simulink model "afe"  (R2026a)
settings: Solver=ode23tb  StopTime=simlength  FixedStep=tc  MaxStep=glb_time.tc
values from neighbouring files (symbols this model uses):
  afe_ctrl = ctrl_afe_setup(glb_time.ts_afe, grid_emu.omega_grid_nom)    [init_model.m]
  afe_pwm_phase_shift_mod1 = 0    [init_model.m]
  CTRPIFF_CLIP_RELEASE = 0.001    [init_model.m]
  glb_time = timing_setup(fpwm_afe, trgo_afe, fpwm_inv, trgo_inv, fpwm_single_phase_inv, trgo_single_phase_inv, fpwm_dab, trgo_dab,      fpwm_psfbc, trgo_psfbc, fpwm_isop_rail, trgo_isop_rail, fpwm_cllc, trgo_cllc, t_measure, tc_factor, tc_decimation, delay_pwm, dead_time_afe,      dead_time_inv, dead_time_single_phase_inv, dead_time_dab, dead_time_psfbc, dead_time_isop_rail, dead_time_cllc)    [init_model.m]
  grid_emu = grid_three_phase_emulator('Dyn11', delta_star, grid_nominal_power, application_voltage, us1, us2, fgrid,                  eq_grid_inductance, eq_grid_resistance, eta, ucc, i1m, p_iron, n1, n2, core_area, core_length, mur,                  up_xi_pu_ref, up_eta_pu_ref, un_xi_pu_ref, un_eta_pu_ref)    [init_model.m]
  heatsink = liquid_cooled_plate_2kw_setup(weight, no_weight, cp_al, heat_capacity_hs, thermal_conductivity_al,      Rth_switch_HA, Rth_mosfet_HA, Rth_diode_HA, Tambient, DThs_init)    [init_model.m]
  ki_align = 18    [init_model.m]
  kp_align = 0.25    [init_model.m]
  lim_down_align = -0.05    [init_model.m]
  lim_up_align = 0.05    [init_model.m]
  psm_ctrl = ctrl_pmsm_setup(glb_time.ts_inv, psm.omega_bez, u_psm_scale, psm.Jm_norm)    [init_model.m]
  Tambient = 40    [init_model.m]
  time_gain_afe_module_1 = 1.0002    [init_model.m]
  time_gain_inv_module_2 = 1.001    [init_model.m]
  u_cm_comp_mod1 = 0    [init_model.m]
undefined symbols (not defined in the file or in its folder): hwdata, igbt, magnitude
libraries: fl_lib x166, nesl_utility x91, igbt_simple_2th_lib x4, single_phase_transformer_lib x3, mos_simple_2th_lib x2, discrete_time_low_pass_filter x1, threephase_inductor_lib x1, dclink_for_two_levels x1, three_phase_pwm_modulator x1, three_phase_voltage_with_frt_emulator x1
(part 5 of 7)

== system afe/afe/afe_dq_mod1/AFE_control/afe_control/grid_voltage_phase_lock_loops/dq_pll_ccaller/first_harmonic_tracker_phase_w ==
  u : Inport
  Bus Selector : BusSelector  OutputSignals=output_pu_hat
  C Caller : CCaller  FunctionName=first_harmonic_tracker_process_simulink  PortSpecificationStruct="%)30     .    B \\   8    (     @         %    \"     D    !     0         %  0 \"0    $    _    07)G3F%M90  4&]R=$YA;64 4V-O<&4     26YD97@     5'EP90      4VEZ90      27-';&]B86P   X    P    !@    @    $          4    (     0    ,    !         !   P!O=70 #@   #     &    \"     0         !0    @    !     P    $         $  # &]U=  .    .     8    (    !          %    \"     $    &     0         0  ...(+4988 chars)"
  Constant : Constant  Value=glb_time.ts_afe
  Constant1 : Constant  Value=4
  Constant4 : Constant  Value=afe_ctrl.fht_grid.omega_fht
  Constant5 : Constant  Value=afe_ctrl.fht_grid.delta_fht
  Constant6 : Constant  Value=afe_ctrl.fht_grid.Ld_fht(1)
  Constant7 : Constant  Value=afe_ctrl.fht_grid.Ld_fht(2)
  Data Type Conversion{1..2,6..9} (6 alike) : DataTypeConversion  OutDataTypeStr=single  SaturateOnIntegerOverflow=off  RndMeth=Floor
  Data Type Conversion3 : DataTypeConversion  OutDataTypeStr=uint8  SaturateOnIntegerOverflow=off  RndMeth=Floor
  Data Type Conversion4 : DataTypeConversion  OutDataTypeStr=double  SaturateOnIntegerOverflow=off  RndMeth=Floor
  Data Type Conversion5 : DataTypeConversion  OutDataTypeStr=uint8  SaturateOnIntegerOverflow=off  RndMeth=Floor
  Step : Step  Time=0.0125  InitialValue=1  FinalValue=0
  u_hat : Outport
  wires:
  Data Type Conversion4/1 -> u_hat/1
  Data Type Conversion3/1 -> C Caller/1
  Data Type Conversion1/1 -> C Caller/3
  Data Type Conversion2/1 -> C Caller/2
  C Caller/1 -> Bus Selector/1
  Bus Selector/1 -> Data Type Conversion4/1  "<output_pu_hat>"
  Step/1 -> Data Type Conversion3/1
  u/1 -> Data Type Conversion2/1
  Constant/1 -> Data Type Conversion1/1
  Constant1/1 -> Data Type Conversion5/1
  Constant4/1 -> Data Type Conversion6/1
  Constant6/1 -> Data Type Conversion8/1
  Constant7/1 -> Data Type Conversion9/1
  Constant5/1 -> Data Type Conversion7/1
  Data Type Conversion5/1 -> C Caller/8
  Data Type Conversion6/1 -> C Caller/4
  Data Type Conversion7/1 -> C Caller/5
  Data Type Conversion8/1 -> C Caller/6
  Data Type Conversion9/1 -> C Caller/7

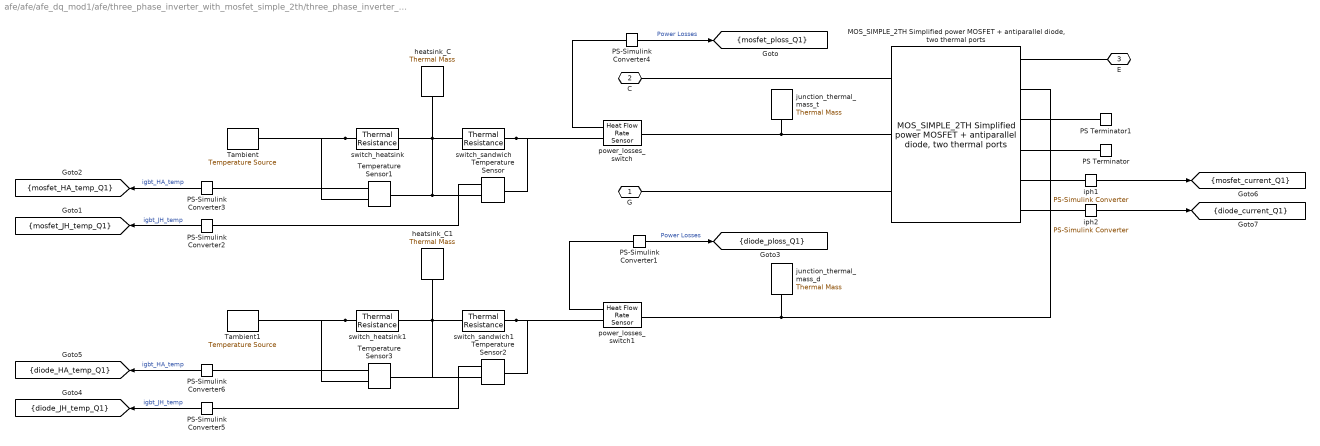
== system afe/afe/afe_dq_mod1/afe/three_phase_inverter_with_mosfet_simple_2th/three_phase_inverter_with_mosfet_simple_2th/mosfet_simple_1/MOSFET_simple ==
  "MOS_SIMPLE_2TH Simplified power MOSFET + antiparallel diode, two thermal ports" : mos_simple_2th_lib/MOS_SIMPLE_2TH Simplified power MOSFET + antiparallel diode, two thermal ports  Rds_on=rds_on_m Ohm  alpha_R=0 1/K  Tj_ref=398.15 K  Roff=1e7 Ohm  Vf=1.0 V  Rd=2.5e-3 Ohm  two_die=1  Eon_ref=Eon_m J  Eoff_ref=Eoff_m J  Err_ref=Err_m J  Iref=Ic_ref_m A  Vref=Vdc_ref_m V  ki=1  kv=1  Vth_off=50 V  Vth_on=25 V  V_sm=10 V  tau_s=100e-9 s  tau_v=10e-6 s  tau_p=50e-6 s  i_eps=1e-3 A  v_eps=1e-3 V  v_specify=off  v_priority=None  v=0 V  v_nominal_specify=off  v_nominal_value=1  v_nominal_unit=V  i_specify=off  i_priority=None  i=0 A  i_nominal_specify=off  i_nominal_value=1  i_nominal_unit=A  ich_specify=off  ich_priority=None  ich=0 A  ich_nominal_specify=off  ich_nominal_value=1  ich_nominal_unit=A  ichp_specify=off  ichp_priority=None  ichp=0 A  ichp_nominal_specify=off  ichp_nominal_value=1  ichp_nominal_unit=A  idio_specify=off  idio_priority=None  idio=0 A  idio_nominal_specify=off  idio_nominal_value=1  idio_nominal_unit=A  vfd_specify=off  vfd_priority=None  vfd=0 V  vfd_nominal_specify=off  vfd_nominal_value=1  vfd_nominal_unit=V  ith_specify=off  ith_priority=None  ith=0 A  ith_nominal_specify=off  ith_nominal_value=1  ith_nominal_unit=A  idh_specify=off  idh_priority=None  idh=0 A  idh_nominal_specify=off  idh_nominal_value=1  idh_nominal_unit=A  vbl_specify=off  vbl_priority=None  vbl=600 V  vbl_nominal_specify=off  vbl_nominal_value=1  vbl_nominal_unit=V  hb_specify=off  hb_priority=None  hb=0  hb_nominal_specify=off  hb_nominal_value=1  hb_nominal_unit=1  Gch_specify=off  Gch_priority=None  Gch=0 S  Gch_nominal_specify=off  Gch_nominal_value=1  Gch_nominal_unit=S  Rds_specify=off  Rds_priority=None  Rds=1e-3 Ohm  Rds_nominal_specify=off  Rds_nominal_value=1  Rds_nominal_unit=Ohm  xr_specify=off  xr_priority=None  xr=1  xr_nominal_specify=off  xr_nominal_value=1  xr_nominal_unit=1  Eot_specify=off  Eot_priority=None  Eot=0 J  Eot_nominal_specify=off  Eot_nominal_value=1  Eot_nominal_unit=J  Eod_specify=off  Eod_priority=None  Eod=0 J  Eod_nominal_specify=off  Eod_nominal_value=1  Eod_nominal_unit=J  Pswt_specify=off  Pswt_priority=None  Pswt=0 W  Pswt_nominal_specify=off  Pswt_nominal_value=1  Pswt_nominal_unit=W  Pswd_specify=off  Pswd_priority=None  Pswd=0 W  Pswd_nominal_specify=off  Pswd_nominal_value=1  Pswd_nominal_unit=W  Pct_specify=off  Pct_priority=None  Pct=0 W  Pct_nominal_specify=off  Pct_nominal_value=1  Pct_nominal_unit=W  Pcd_specify=off  Pcd_priority=None  Pcd=0 W  Pcd_nominal_specify=off  Pcd_nominal_value=1  Pcd_nominal_unit=W  Qt_specify=off  Qt_priority=None  Qt=0 W  Qt_nominal_specify=off  Qt_nominal_value=1  Qt_nominal_unit=W  Qd_specify=off  Qd_priority=None  Qd=0 W  Qd_nominal_specify=off  Qd_nominal_value=1  Qd_nominal_unit=W  Eqt_specify=off  Eqt_priority=None  Eqt=0 J  Eqd_specify=off  Eqd_priority=None  Eqd=0 J
  PS Terminator : fl_lib/Physical Signals/Sinks/PS Terminator
  PS Terminator1 : fl_lib/Physical Signals/Sinks/PS Terminator
  PS-Simulink Converter1 : nesl_utility/PS-Simulink Converter  PhysicalDomain=network_engine_domain  SubClassName=ps_output  LeftPortType=input  RightPortType=output  PseudoPeriodic=off  Frequencies=[]  VectorFormat=1-D array  Unit=J/s  AffineConversion=off
  PS-Simulink Converter{2..3,5..6} (4 alike) : nesl_utility/PS-Simulink Converter  PhysicalDomain=network_engine_domain  SubClassName=ps_output  LeftPortType=input  RightPortType=output  PseudoPeriodic=off  Frequencies=[]  VectorFormat=1-D array  Unit=degC  AffineConversion=off
  PS-Simulink Converter4 : nesl_utility/PS-Simulink Converter  PhysicalDomain=network_engine_domain  SubClassName=ps_output  LeftPortType=input  RightPortType=output  PseudoPeriodic=off  Frequencies=[]  VectorFormat=1-D array  Unit=J/s  AffineConversion=off
  Tambient : fl_lib/Thermal/Thermal Sources/Temperature Source  temperature=Tambient_m degC
  Tambient1 : fl_lib/Thermal/Thermal Sources/Temperature Source  temperature=Tambient_m degC
  Temperature Sensor{,1..3} (4 alike) : fl_lib/Thermal/Thermal Sensors/Temperature Sensor  temperature_measure=foundation.enum.MeasurementReference.difference
  heatsink_C : fl_lib/Thermal/Thermal Elements/Thermal Mass  mass_type=foundation.enum.constant_variable.constant  mass=mass_heatsink_m kg  sp_heat=specific_heat_m J/(K*kg)  mass_min=1e-6 kg  num_ports=foundation.enum.numPorts2.one  m_specify=off  m_priority=High  m=1 kg  m_nominal_specify=off  m_nominal_value=1  m_nominal_unit=kg  T_specify=on  T_priority=High  T=Tambient_m degC  T_nominal_specify=off  T_nominal_value=1  T_nominal_unit=K  Q_specify=off  Q_priority=High  Q=0 W  Q_nominal_specify=off  Q_nominal_value=1  Q_nominal_unit=W
  heatsink_C1 : fl_lib/Thermal/Thermal Elements/Thermal Mass  mass_type=foundation.enum.constant_variable.constant  mass=mass_heatsink_m kg  sp_heat=specific_heat_m J/(K*kg)  mass_min=1e-6 kg  num_ports=foundation.enum.numPorts2.one  m_specify=off  m_priority=High  m=1 kg  m_nominal_specify=off  m_nominal_value=1  m_nominal_unit=kg  T_specify=on  T_priority=High  T=Tambient_m degC  T_nominal_specify=off  T_nominal_value=1  T_nominal_unit=K  Q_specify=off  Q_priority=High  Q=0 W  Q_nominal_specify=off  Q_nominal_value=1  Q_nominal_unit=W
  iph1 : nesl_utility/PS-Simulink Converter  PhysicalDomain=network_engine_domain  SubClassName=ps_output  LeftPortType=input  RightPortType=output  PseudoPeriodic=off  Frequencies=[]  VectorFormat=1-D array  Unit=A  AffineConversion=off
  iph2 : nesl_utility/PS-Simulink Converter  PhysicalDomain=network_engine_domain  SubClassName=ps_output  LeftPortType=input  RightPortType=output  PseudoPeriodic=off  Frequencies=[]  VectorFormat=1-D array  Unit=A  AffineConversion=off
  junction_thermal_mass_d : fl_lib/Thermal/Thermal Elements/Thermal Mass  mass_type=foundation.enum.constant_variable.constant  mass=JunctionTermalMass_m/specific_heat_m kg  sp_heat=specific_heat_m J/(K*kg)  mass_min=1e-6 kg  num_ports=foundation.enum.numPorts2.one  m_specify=off  m_priority=High  m=1 kg  m_nominal_specify=off  m_nominal_value=1  m_nominal_unit=kg  T_specify=on  T_priority=High  T=Tambient_m degC  T_nominal_specify=off  T_nominal_value=1  T_nominal_unit=K  Q_specify=off  Q_priority=High  Q=0 W  Q_nominal_specify=off  Q_nominal_value=1  Q_nominal_unit=W
  junction_thermal_mass_t : fl_lib/Thermal/Thermal Elements/Thermal Mass  mass_type=foundation.enum.constant_variable.constant  mass=JunctionTermalMass_m/specific_heat_m kg  sp_heat=specific_heat_m J/(K*kg)  mass_min=1e-6 kg  num_ports=foundation.enum.numPorts2.one  m_specify=off  m_priority=High  m=1 kg  m_nominal_specify=off  m_nominal_value=1  m_nominal_unit=kg  T_specify=on  T_priority=High  T=Tambient_m degC  T_nominal_specify=off  T_nominal_value=1  T_nominal_unit=K  Q_specify=off  Q_priority=High  Q=0 W  Q_nominal_specify=off  Q_nominal_value=1  Q_nominal_unit=W
  power_losses_switch : fl_lib/Thermal/Thermal Sensors/Heat Flow Rate Sensor
  power_losses_switch1 : fl_lib/Thermal/Thermal Sensors/Heat Flow Rate Sensor
  switch_heatsink : fl_lib/Thermal/Thermal Elements/Thermal Resistance  resistance=rth_switch_HA_m K/W  T_specify=off  T_priority=High  T=0 deltadegC  T_nominal_specify=off  T_nominal_value=1  T_nominal_unit=K  Q_specify=off  Q_priority=None  Q=0 W  Q_nominal_specify=off  Q_nominal_value=1  Q_nominal_unit=W
  switch_heatsink1 : fl_lib/Thermal/Thermal Elements/Thermal Resistance  resistance=rth_diode_HA_m K/W  T_specify=off  T_priority=High  T=0 deltadegC  T_nominal_specify=off  T_nominal_value=1  T_nominal_unit=K  Q_specify=off  Q_priority=None  Q=0 W  Q_nominal_specify=off  Q_nominal_value=1  Q_nominal_unit=W
  switch_sandwich : fl_lib/Thermal/Thermal Elements/Thermal Resistance  resistance=rth_switch_JH_m K/W  T_specify=off  T_priority=High  T=0 degC  T_nominal_specify=off  T_nominal_value=1  T_nominal_unit=K  Q_specify=off  Q_priority=None  Q=0 W  Q_nominal_specify=off  Q_nominal_value=1  Q_nominal_unit=W
  switch_sandwich1 : fl_lib/Thermal/Thermal Elements/Thermal Resistance  resistance=rth_diode_JH_m K/W  T_specify=off  T_priority=High  T=0 degC  T_nominal_specify=off  T_nominal_value=1  T_nominal_unit=K  Q_specify=off  Q_priority=None  Q=0 W  Q_nominal_specify=off  Q_nominal_value=1  Q_nominal_unit=W
  G : PMIOPort  Side=Left
  C : PMIOPort  Port=2  Side=Left
  E : PMIOPort  Port=3  Side=Right
  tag scope: diode_HA_temp_Q1=scoped, diode_JH_temp_Q1=scoped, diode_current_Q1=scoped, diode_ploss_Q1=scoped, mosfet_HA_temp_Q1=scoped, mosfet_JH_temp_Q1=scoped, mosfet_current_Q1=scoped, mosfet_ploss_Q1=scoped
  wires:
  PS-Simulink Converter3/1 -> [mosfet_HA_temp_Q1]  "igbt_HA_temp"
  PS-Simulink Converter4/1 -> [mosfet_ploss_Q1]  "Power Losses"
  PS-Simulink Converter2/1 -> [mosfet_JH_temp_Q1]  "igbt_JH_temp"
  PS-Simulink Converter1/1 -> [diode_ploss_Q1]  "Power Losses"
  PS-Simulink Converter5/1 -> [diode_JH_temp_Q1]  "igbt_JH_temp"
  PS-Simulink Converter6/1 -> [diode_HA_temp_Q1]  "igbt_HA_temp"
  iph1/1 -> [mosfet_current_Q1]
  iph2/1 -> [diode_current_Q1]
  connections:
  Temperature Sensor/RConn2 -- PS-Simulink Converter2/LConn1
  junction_thermal_mass_t/LConn1 -- "MOS_SIMPLE_2TH Simplified power MOSFET + antiparallel diode, two thermal ports"/LConn2 -- power_losses_switch/LConn1
  Temperature Sensor1/RConn2 -- PS-Simulink Converter3/LConn1
  Temperature Sensor1/LConn1 -- Temperature Sensor/RConn1 -- switch_heatsink/LConn1 -- heatsink_C/LConn1 -- switch_sandwich/RConn1
  switch_heatsink/RConn1 -- Tambient/LConn1 -- Temperature Sensor1/RConn1
  switch_sandwich/LConn1 -- power_losses_switch/RConn2 -- Temperature Sensor/LConn1
  "MOS_SIMPLE_2TH Simplified power MOSFET + antiparallel diode, two thermal ports"/RConn1 -- E/RConn1
  "MOS_SIMPLE_2TH Simplified power MOSFET + antiparallel diode, two thermal ports"/LConn1 -- C/RConn1
  "MOS_SIMPLE_2TH Simplified power MOSFET + antiparallel diode, two thermal ports"/LConn3 -- G/RConn1
  switch_heatsink1/LConn1 -- switch_sandwich1/RConn1 -- heatsink_C1/LConn1 -- Temperature Sensor2/RConn1 -- Temperature Sensor3/LConn1
  switch_heatsink1/RConn1 -- Temperature Sensor3/RConn1 -- Tambient1/LConn1
  switch_sandwich1/LConn1 -- Temperature Sensor2/LConn1 -- power_losses_switch1/RConn2
  Temperature Sensor3/RConn2 -- PS-Simulink Converter6/LConn1
  Temperature Sensor2/RConn2 -- PS-Simulink Converter5/LConn1
  power_losses_switch1/LConn1 -- "MOS_SIMPLE_2TH Simplified power MOSFET + antiparallel diode, two thermal ports"/RConn2 -- junction_thermal_mass_d/LConn1
  "MOS_SIMPLE_2TH Simplified power MOSFET + antiparallel diode, two thermal ports"/RConn5 -- iph1/LConn1
  "MOS_SIMPLE_2TH Simplified power MOSFET + antiparallel diode, two thermal ports"/RConn6 -- iph2/LConn1
  "MOS_SIMPLE_2TH Simplified power MOSFET + antiparallel diode, two thermal ports"/RConn3 -- PS Terminator1/LConn1
  "MOS_SIMPLE_2TH Simplified power MOSFET + antiparallel diode, two thermal ports"/RConn4 -- PS Terminator/LConn1
  PS-Simulink Converter4/LConn1 -- power_losses_switch/RConn1
  PS-Simulink Converter1/LConn1 -- power_losses_switch1/RConn1

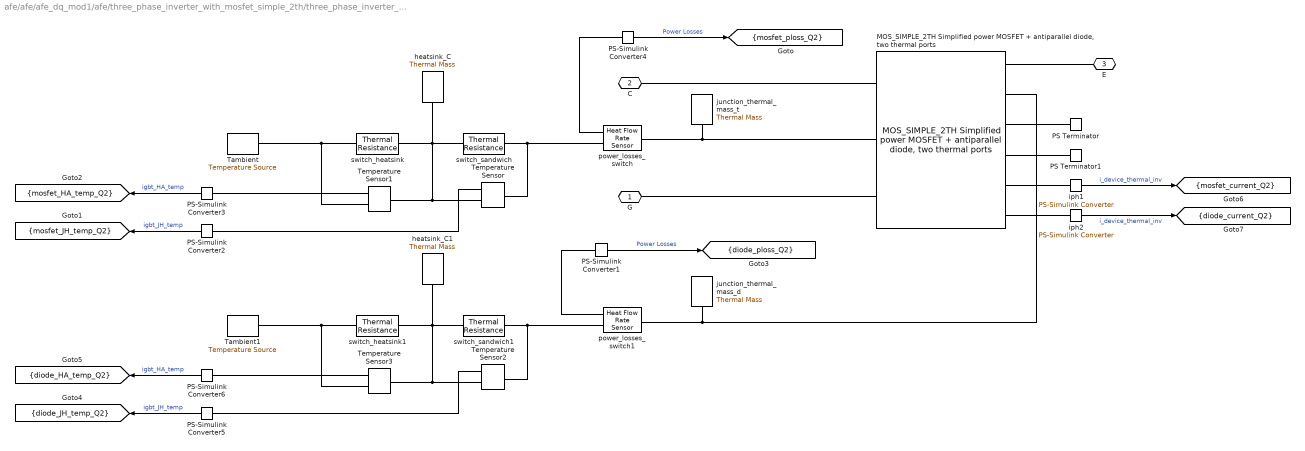
== system afe/afe/afe_dq_mod1/afe/three_phase_inverter_with_mosfet_simple_2th/three_phase_inverter_with_mosfet_simple_2th/mosfet_simple_2/MOSFET_simple ==
  "MOS_SIMPLE_2TH Simplified power MOSFET + antiparallel diode, two thermal ports" : mos_simple_2th_lib/MOS_SIMPLE_2TH Simplified power MOSFET + antiparallel diode, two thermal ports  Rds_on=rds_on_m Ohm  alpha_R=0 1/K  Tj_ref=398.15 K  Roff=1e7 Ohm  Vf=1.0 V  Rd=2.5e-3 Ohm  two_die=1  Eon_ref=Eon_m J  Eoff_ref=Eoff_m J  Err_ref=Err_m J  Iref=Ic_ref_m A  Vref=Vdc_ref_m V  ki=1  kv=1  Vth_off=50 V  Vth_on=25 V  V_sm=10 V  tau_s=100e-9 s  tau_v=10e-6 s  tau_p=50e-6 s  i_eps=1e-3 A  v_eps=1e-3 V  v_specify=off  v_priority=None  v=0 V  v_nominal_specify=off  v_nominal_value=1  v_nominal_unit=V  i_specify=off  i_priority=None  i=0 A  i_nominal_specify=off  i_nominal_value=1  i_nominal_unit=A  ich_specify=off  ich_priority=None  ich=0 A  ich_nominal_specify=off  ich_nominal_value=1  ich_nominal_unit=A  ichp_specify=off  ichp_priority=None  ichp=0 A  ichp_nominal_specify=off  ichp_nominal_value=1  ichp_nominal_unit=A  idio_specify=off  idio_priority=None  idio=0 A  idio_nominal_specify=off  idio_nominal_value=1  idio_nominal_unit=A  vfd_specify=off  vfd_priority=None  vfd=0 V  vfd_nominal_specify=off  vfd_nominal_value=1  vfd_nominal_unit=V  ith_specify=off  ith_priority=None  ith=0 A  ith_nominal_specify=off  ith_nominal_value=1  ith_nominal_unit=A  idh_specify=off  idh_priority=None  idh=0 A  idh_nominal_specify=off  idh_nominal_value=1  idh_nominal_unit=A  vbl_specify=off  vbl_priority=None  vbl=600 V  vbl_nominal_specify=off  vbl_nominal_value=1  vbl_nominal_unit=V  hb_specify=off  hb_priority=None  hb=0  hb_nominal_specify=off  hb_nominal_value=1  hb_nominal_unit=1  Gch_specify=off  Gch_priority=None  Gch=0 S  Gch_nominal_specify=off  Gch_nominal_value=1  Gch_nominal_unit=S  Rds_specify=off  Rds_priority=None  Rds=1e-3 Ohm  Rds_nominal_specify=off  Rds_nominal_value=1  Rds_nominal_unit=Ohm  xr_specify=off  xr_priority=None  xr=1  xr_nominal_specify=off  xr_nominal_value=1  xr_nominal_unit=1  Eot_specify=off  Eot_priority=None  Eot=0 J  Eot_nominal_specify=off  Eot_nominal_value=1  Eot_nominal_unit=J  Eod_specify=off  Eod_priority=None  Eod=0 J  Eod_nominal_specify=off  Eod_nominal_value=1  Eod_nominal_unit=J  Pswt_specify=off  Pswt_priority=None  Pswt=0 W  Pswt_nominal_specify=off  Pswt_nominal_value=1  Pswt_nominal_unit=W  Pswd_specify=off  Pswd_priority=None  Pswd=0 W  Pswd_nominal_specify=off  Pswd_nominal_value=1  Pswd_nominal_unit=W  Pct_specify=off  Pct_priority=None  Pct=0 W  Pct_nominal_specify=off  Pct_nominal_value=1  Pct_nominal_unit=W  Pcd_specify=off  Pcd_priority=None  Pcd=0 W  Pcd_nominal_specify=off  Pcd_nominal_value=1  Pcd_nominal_unit=W  Qt_specify=off  Qt_priority=None  Qt=0 W  Qt_nominal_specify=off  Qt_nominal_value=1  Qt_nominal_unit=W  Qd_specify=off  Qd_priority=None  Qd=0 W  Qd_nominal_specify=off  Qd_nominal_value=1  Qd_nominal_unit=W  Eqt_specify=off  Eqt_priority=None  Eqt=0 J  Eqd_specify=off  Eqd_priority=None  Eqd=0 J
  PS Terminator : fl_lib/Physical Signals/Sinks/PS Terminator
  PS Terminator1 : fl_lib/Physical Signals/Sinks/PS Terminator
  PS-Simulink Converter1 : nesl_utility/PS-Simulink Converter  PhysicalDomain=network_engine_domain  SubClassName=ps_output  LeftPortType=input  RightPortType=output  PseudoPeriodic=off  Frequencies=[]  VectorFormat=1-D array  Unit=J/s  AffineConversion=off
  PS-Simulink Converter{2..3,5..6} (4 alike) : nesl_utility/PS-Simulink Converter  PhysicalDomain=network_engine_domain  SubClassName=ps_output  LeftPortType=input  RightPortType=output  PseudoPeriodic=off  Frequencies=[]  VectorFormat=1-D array  Unit=degC  AffineConversion=off
  PS-Simulink Converter4 : nesl_utility/PS-Simulink Converter  PhysicalDomain=network_engine_domain  SubClassName=ps_output  LeftPortType=input  RightPortType=output  PseudoPeriodic=off  Frequencies=[]  VectorFormat=1-D array  Unit=J/s  AffineConversion=off
  Tambient : fl_lib/Thermal/Thermal Sources/Temperature Source  temperature=Tambient_m degC
  Tambient1 : fl_lib/Thermal/Thermal Sources/Temperature Source  temperature=Tambient_m degC
  Temperature Sensor{,1..3} (4 alike) : fl_lib/Thermal/Thermal Sensors/Temperature Sensor  temperature_measure=foundation.enum.MeasurementReference.difference
  heatsink_C : fl_lib/Thermal/Thermal Elements/Thermal Mass  mass_type=foundation.enum.constant_variable.constant  mass=mass_heatsink_m kg  sp_heat=specific_heat_m J/(K*kg)  mass_min=1e-6 kg  num_ports=foundation.enum.numPorts2.one  m_specify=off  m_priority=High  m=1 kg  m_nominal_specify=off  m_nominal_value=1  m_nominal_unit=kg  T_specify=on  T_priority=High  T=Tambient_m degC  T_nominal_specify=off  T_nominal_value=1  T_nominal_unit=K  Q_specify=off  Q_priority=High  Q=0 W  Q_nominal_specify=off  Q_nominal_value=1  Q_nominal_unit=W
  heatsink_C1 : fl_lib/Thermal/Thermal Elements/Thermal Mass  mass_type=foundation.enum.constant_variable.constant  mass=mass_heatsink_m kg  sp_heat=specific_heat_m J/(K*kg)  mass_min=1e-6 kg  num_ports=foundation.enum.numPorts2.one  m_specify=off  m_priority=High  m=1 kg  m_nominal_specify=off  m_nominal_value=1  m_nominal_unit=kg  T_specify=on  T_priority=High  T=Tambient_m degC  T_nominal_specify=off  T_nominal_value=1  T_nominal_unit=K  Q_specify=off  Q_priority=High  Q=0 W  Q_nominal_specify=off  Q_nominal_value=1  Q_nominal_unit=W
  iph1 : nesl_utility/PS-Simulink Converter  PhysicalDomain=network_engine_domain  SubClassName=ps_output  LeftPortType=input  RightPortType=output  PseudoPeriodic=off  Frequencies=[]  VectorFormat=1-D array  Unit=A  AffineConversion=off
  iph2 : nesl_utility/PS-Simulink Converter  PhysicalDomain=network_engine_domain  SubClassName=ps_output  LeftPortType=input  RightPortType=output  PseudoPeriodic=off  Frequencies=[]  VectorFormat=1-D array  Unit=A  AffineConversion=off
  junction_thermal_mass_d : fl_lib/Thermal/Thermal Elements/Thermal Mass  mass_type=foundation.enum.constant_variable.constant  mass=JunctionTermalMass_m/specific_heat_m kg  sp_heat=specific_heat_m J/(K*kg)  mass_min=1e-6 kg  num_ports=foundation.enum.numPorts2.one  m_specify=off  m_priority=High  m=1 kg  m_nominal_specify=off  m_nominal_value=1  m_nominal_unit=kg  T_specify=on  T_priority=High  T=Tambient_m degC  T_nominal_specify=off  T_nominal_value=1  T_nominal_unit=K  Q_specify=off  Q_priority=High  Q=0 W  Q_nominal_specify=off  Q_nominal_value=1  Q_nominal_unit=W
  junction_thermal_mass_t : fl_lib/Thermal/Thermal Elements/Thermal Mass  mass_type=foundation.enum.constant_variable.constant  mass=JunctionTermalMass_m/specific_heat_m kg  sp_heat=specific_heat_m J/(K*kg)  mass_min=1e-6 kg  num_ports=foundation.enum.numPorts2.one  m_specify=off  m_priority=High  m=1 kg  m_nominal_specify=off  m_nominal_value=1  m_nominal_unit=kg  T_specify=on  T_priority=High  T=Tambient_m degC  T_nominal_specify=off  T_nominal_value=1  T_nominal_unit=K  Q_specify=off  Q_priority=High  Q=0 W  Q_nominal_specify=off  Q_nominal_value=1  Q_nominal_unit=W
  power_losses_switch : fl_lib/Thermal/Thermal Sensors/Heat Flow Rate Sensor
  power_losses_switch1 : fl_lib/Thermal/Thermal Sensors/Heat Flow Rate Sensor
  switch_heatsink : fl_lib/Thermal/Thermal Elements/Thermal Resistance  resistance=rth_switch_HA_m K/W  T_specify=off  T_priority=High  T=0 deltadegC  T_nominal_specify=off  T_nominal_value=1  T_nominal_unit=K  Q_specify=off  Q_priority=None  Q=0 W  Q_nominal_specify=off  Q_nominal_value=1  Q_nominal_unit=W
  switch_heatsink1 : fl_lib/Thermal/Thermal Elements/Thermal Resistance  resistance=rth_diode_HA_m K/W  T_specify=off  T_priority=High  T=0 deltadegC  T_nominal_specify=off  T_nominal_value=1  T_nominal_unit=K  Q_specify=off  Q_priority=None  Q=0 W  Q_nominal_specify=off  Q_nominal_value=1  Q_nominal_unit=W
  switch_sandwich : fl_lib/Thermal/Thermal Elements/Thermal Resistance  resistance=rth_switch_JH_m K/W  T_specify=off  T_priority=High  T=0 degC  T_nominal_specify=off  T_nominal_value=1  T_nominal_unit=K  Q_specify=off  Q_priority=None  Q=0 W  Q_nominal_specify=off  Q_nominal_value=1  Q_nominal_unit=W
  switch_sandwich1 : fl_lib/Thermal/Thermal Elements/Thermal Resistance  resistance=rth_diode_JH_m K/W  T_specify=off  T_priority=High  T=0 degC  T_nominal_specify=off  T_nominal_value=1  T_nominal_unit=K  Q_specify=off  Q_priority=None  Q=0 W  Q_nominal_specify=off  Q_nominal_value=1  Q_nominal_unit=W
  G : PMIOPort  Side=Left
  C : PMIOPort  Port=2  Side=Left
  E : PMIOPort  Port=3  Side=Right
  tag scope: diode_HA_temp_Q2=scoped, diode_JH_temp_Q2=scoped, diode_current_Q2=scoped, diode_ploss_Q2=scoped, mosfet_HA_temp_Q2=scoped, mosfet_JH_temp_Q2=scoped, mosfet_current_Q2=scoped, mosfet_ploss_Q2=scoped
  wires:
  iph2/1 -> [diode_current_Q2]  "i_device_thermal_inv"
  iph1/1 -> [mosfet_current_Q2]  "i_device_thermal_inv"
  PS-Simulink Converter6/1 -> [diode_HA_temp_Q2]  "igbt_HA_temp"
  PS-Simulink Converter5/1 -> [diode_JH_temp_Q2]  "igbt_JH_temp"
  PS-Simulink Converter1/1 -> [diode_ploss_Q2]  "Power Losses"
  PS-Simulink Converter2/1 -> [mosfet_JH_temp_Q2]  "igbt_JH_temp"
  PS-Simulink Converter4/1 -> [mosfet_ploss_Q2]  "Power Losses"
  PS-Simulink Converter3/1 -> [mosfet_HA_temp_Q2]  "igbt_HA_temp"
  connections:
  "MOS_SIMPLE_2TH Simplified power MOSFET + antiparallel diode, two thermal ports"/RConn6 -- iph2/LConn1
  "MOS_SIMPLE_2TH Simplified power MOSFET + antiparallel diode, two thermal ports"/RConn5 -- iph1/LConn1
  power_losses_switch1/LConn1 -- "MOS_SIMPLE_2TH Simplified power MOSFET + antiparallel diode, two thermal ports"/RConn2 -- junction_thermal_mass_d/LConn1
  Temperature Sensor2/RConn2 -- PS-Simulink Converter5/LConn1
  Temperature Sensor3/RConn2 -- PS-Simulink Converter6/LConn1
  Temperature Sensor2/LConn1 -- switch_sandwich1/LConn1 -- power_losses_switch1/RConn2
  Temperature Sensor3/RConn1 -- switch_heatsink1/RConn1 -- Tambient1/LConn1
  Temperature Sensor3/LConn1 -- Temperature Sensor2/RConn1 -- switch_sandwich1/RConn1 -- switch_heatsink1/LConn1 -- heatsink_C1/LConn1
  "MOS_SIMPLE_2TH Simplified power MOSFET + antiparallel diode, two thermal ports"/LConn3 -- G/RConn1
  "MOS_SIMPLE_2TH Simplified power MOSFET + antiparallel diode, two thermal ports"/LConn1 -- C/RConn1
  "MOS_SIMPLE_2TH Simplified power MOSFET + antiparallel diode, two thermal ports"/RConn1 -- E/RConn1
  Temperature Sensor/LConn1 -- power_losses_switch/RConn2 -- switch_sandwich/LConn1
  Temperature Sensor1/RConn1 -- Tambient/LConn1 -- switch_heatsink/RConn1
  Temperature Sensor/RConn1 -- Temperature Sensor1/LConn1 -- switch_sandwich/RConn1 -- heatsink_C/LConn1 -- switch_heatsink/LConn1
  Temperature Sensor1/RConn2 -- PS-Simulink Converter3/LConn1
  junction_thermal_mass_t/LConn1 -- "MOS_SIMPLE_2TH Simplified power MOSFET + antiparallel diode, two thermal ports"/LConn2 -- power_losses_switch/LConn1
  Temperature Sensor/RConn2 -- PS-Simulink Converter2/LConn1
  "MOS_SIMPLE_2TH Simplified power MOSFET + antiparallel diode, two thermal ports"/RConn4 -- PS Terminator1/LConn1
  "MOS_SIMPLE_2TH Simplified power MOSFET + antiparallel diode, two thermal ports"/RConn3 -- PS Terminator/LConn1
  PS-Simulink Converter4/LConn1 -- power_losses_switch/RConn1
  PS-Simulink Converter1/LConn1 -- power_losses_switch1/RConn1

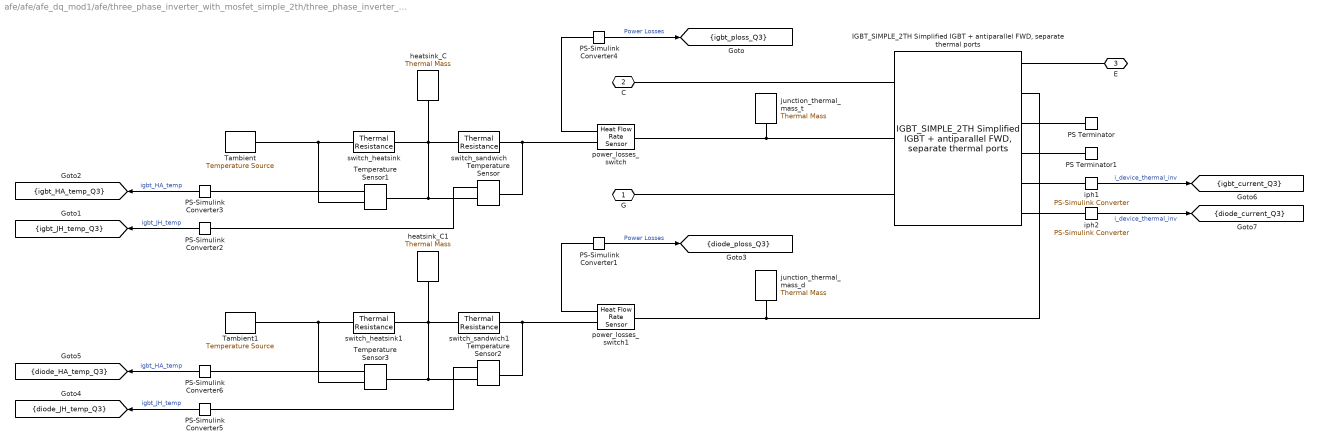
== system afe/afe/afe_dq_mod1/afe/three_phase_inverter_with_mosfet_simple_2th/three_phase_inverter_with_mosfet_simple_2th/mosfet_simple_3/IGBT_simple ==
  "IGBT_SIMPLE_2TH Simplified IGBT + antiparallel FWD, separate thermal ports" : igbt_simple_2th_lib/IGBT_SIMPLE_2TH Simplified IGBT + antiparallel FWD, separate thermal ports  Vce_sat=vce_sat_m V  Vf=v_gamma_m V  Vth=Vth_gate_m V  Vhyst=Vth_gate_hyst_m V  Eon_ref=Eon_m mJ  Eoff_ref=Eoff_m mJ  Err_ref=Err_m mJ  Ic_ref=Ic_ref_m A  Vdc_ref=Vdc_ref_m V  V_rr_th=Vblock_Errf_m V  Ron=rce_on_m mOhm  Rd=rd_on_m mOhm  Goff=Gce_off_m 1/Ohm  tau_s=time_constant_edge_m us  tau_p=time_constant_ploss_m us  i_specify=off  i_priority=None  i=0 A  i_nominal_specify=off  i_nominal_value=1  i_nominal_unit=A  v_specify=off  v_priority=None  v=0 V  v_nominal_specify=off  v_nominal_value=1  v_nominal_unit=V  i_t_specify=off  i_t_priority=None  i_t=0 A  i_t_nominal_specify=off  i_t_nominal_value=1  i_t_nominal_unit=A  i_d_specify=off  i_d_priority=None  i_d=0 A  i_d_nominal_specify=off  i_d_nominal_value=1  i_d_nominal_unit=A  i_h_specify=off  i_h_priority=None  i_h=0 A  i_h_nominal_specify=off  i_h_nominal_value=1  i_h_nominal_unit=A  i_dh_specify=off  i_dh_priority=None  i_dh=0 A  i_dh_nominal_specify=off  i_dh_nominal_value=1  i_dh_nominal_unit=A  v_h_specify=off  v_h_priority=None  v_h=0 V  v_h_nominal_specify=off  v_h_nominal_value=1  v_h_nominal_unit=V  E_lpt_specify=off  E_lpt_priority=None  E_lpt=0 J  E_lpt_nominal_specify=off  E_lpt_nominal_value=1  E_lpt_nominal_unit=J  E_lpd_specify=off  E_lpd_priority=None  E_lpd=0 J  E_lpd_nominal_specify=off  E_lpd_nominal_value=1  E_lpd_nominal_unit=J  Qt_specify=off  Qt_priority=None  Qt=0 W  Qt_nominal_specify=off  Qt_nominal_value=1  Qt_nominal_unit=W  Qd_specify=off  Qd_priority=None  Qd=0 W  Qd_nominal_specify=off  Qd_nominal_value=1  Qd_nominal_unit=W  E_t_specify=off  E_t_priority=None  E_t=0 J  E_d_specify=off  E_d_priority=None  E_d=0 J
  PS Terminator : fl_lib/Physical Signals/Sinks/PS Terminator
  PS Terminator1 : fl_lib/Physical Signals/Sinks/PS Terminator
  PS-Simulink Converter1 : nesl_utility/PS-Simulink Converter  PhysicalDomain=network_engine_domain  SubClassName=ps_output  LeftPortType=input  RightPortType=output  PseudoPeriodic=off  Frequencies=[]  VectorFormat=1-D array  Unit=J/s  AffineConversion=off
  PS-Simulink Converter{2..3,5..6} (4 alike) : nesl_utility/PS-Simulink Converter  PhysicalDomain=network_engine_domain  SubClassName=ps_output  LeftPortType=input  RightPortType=output  PseudoPeriodic=off  Frequencies=[]  VectorFormat=1-D array  Unit=degC  AffineConversion=off
  PS-Simulink Converter4 : nesl_utility/PS-Simulink Converter  PhysicalDomain=network_engine_domain  SubClassName=ps_output  LeftPortType=input  RightPortType=output  PseudoPeriodic=off  Frequencies=[]  VectorFormat=1-D array  Unit=J/s  AffineConversion=off
  Tambient : fl_lib/Thermal/Thermal Sources/Temperature Source  temperature=Tambient_m degC
  Tambient1 : fl_lib/Thermal/Thermal Sources/Temperature Source  temperature=Tambient_m degC
  Temperature Sensor{,1..3} (4 alike) : fl_lib/Thermal/Thermal Sensors/Temperature Sensor  temperature_measure=foundation.enum.MeasurementReference.difference
  heatsink_C : fl_lib/Thermal/Thermal Elements/Thermal Mass  mass_type=foundation.enum.constant_variable.constant  mass=mass_heatsink_m kg  sp_heat=specific_heat_m J/(K*kg)  mass_min=1e-6 kg  num_ports=foundation.enum.numPorts2.one  m_specify=off  m_priority=High  m=1 kg  m_nominal_specify=off  m_nominal_value=1  m_nominal_unit=kg  T_specify=on  T_priority=High  T=Tambient_m degC  T_nominal_specify=off  T_nominal_value=1  T_nominal_unit=K  Q_specify=off  Q_priority=High  Q=0 W  Q_nominal_specify=off  Q_nominal_value=1  Q_nominal_unit=W
  heatsink_C1 : fl_lib/Thermal/Thermal Elements/Thermal Mass  mass_type=foundation.enum.constant_variable.constant  mass=mass_heatsink_m kg  sp_heat=specific_heat_m J/(K*kg)  mass_min=1e-6 kg  num_ports=foundation.enum.numPorts2.one  m_specify=off  m_priority=High  m=1 kg  m_nominal_specify=off  m_nominal_value=1  m_nominal_unit=kg  T_specify=on  T_priority=High  T=Tambient_m degC  T_nominal_specify=off  T_nominal_value=1  T_nominal_unit=K  Q_specify=off  Q_priority=High  Q=0 W  Q_nominal_specify=off  Q_nominal_value=1  Q_nominal_unit=W
  iph1 : nesl_utility/PS-Simulink Converter  PhysicalDomain=network_engine_domain  SubClassName=ps_output  LeftPortType=input  RightPortType=output  PseudoPeriodic=off  Frequencies=[]  VectorFormat=1-D array  Unit=A  AffineConversion=off
  iph2 : nesl_utility/PS-Simulink Converter  PhysicalDomain=network_engine_domain  SubClassName=ps_output  LeftPortType=input  RightPortType=output  PseudoPeriodic=off  Frequencies=[]  VectorFormat=1-D array  Unit=A  AffineConversion=off
  junction_thermal_mass_d : fl_lib/Thermal/Thermal Elements/Thermal Mass  mass_type=foundation.enum.constant_variable.constant  mass=JunctionTermalMass_m/specific_heat_m kg  sp_heat=specific_heat_m J/(K*kg)  mass_min=1e-6 kg  num_ports=foundation.enum.numPorts2.one  m_specify=off  m_priority=High  m=1 kg  m_nominal_specify=off  m_nominal_value=1  m_nominal_unit=kg  T_specify=on  T_priority=High  T=Tambient_m degC  T_nominal_specify=off  T_nominal_value=1  T_nominal_unit=K  Q_specify=off  Q_priority=High  Q=0 W  Q_nominal_specify=off  Q_nominal_value=1  Q_nominal_unit=W
  junction_thermal_mass_t : fl_lib/Thermal/Thermal Elements/Thermal Mass  mass_type=foundation.enum.constant_variable.constant  mass=JunctionTermalMass_m/specific_heat_m kg  sp_heat=specific_heat_m J/(K*kg)  mass_min=1e-6 kg  num_ports=foundation.enum.numPorts2.one  m_specify=off  m_priority=High  m=1 kg  m_nominal_specify=off  m_nominal_value=1  m_nominal_unit=kg  T_specify=on  T_priority=High  T=Tambient_m degC  T_nominal_specify=off  T_nominal_value=1  T_nominal_unit=K  Q_specify=off  Q_priority=High  Q=0 W  Q_nominal_specify=off  Q_nominal_value=1  Q_nominal_unit=W
  power_losses_switch : fl_lib/Thermal/Thermal Sensors/Heat Flow Rate Sensor
  power_losses_switch1 : fl_lib/Thermal/Thermal Sensors/Heat Flow Rate Sensor
  switch_heatsink : fl_lib/Thermal/Thermal Elements/Thermal Resistance  resistance=rth_switch_HA_m K/W  T_specify=off  T_priority=High  T=0 deltadegC  T_nominal_specify=off  T_nominal_value=1  T_nominal_unit=K  Q_specify=off  Q_priority=None  Q=0 W  Q_nominal_specify=off  Q_nominal_value=1  Q_nominal_unit=W
  switch_heatsink1 : fl_lib/Thermal/Thermal Elements/Thermal Resistance  resistance=rth_diode_HA_m K/W  T_specify=off  T_priority=High  T=0 deltadegC  T_nominal_specify=off  T_nominal_value=1  T_nominal_unit=K  Q_specify=off  Q_priority=None  Q=0 W  Q_nominal_specify=off  Q_nominal_value=1  Q_nominal_unit=W
  switch_sandwich : fl_lib/Thermal/Thermal Elements/Thermal Resistance  resistance=rth_switch_JH_m K/W  T_specify=off  T_priority=High  T=0 degC  T_nominal_specify=off  T_nominal_value=1  T_nominal_unit=K  Q_specify=off  Q_priority=None  Q=0 W  Q_nominal_specify=off  Q_nominal_value=1  Q_nominal_unit=W
  switch_sandwich1 : fl_lib/Thermal/Thermal Elements/Thermal Resistance  resistance=rth_diode_JH_m K/W  T_specify=off  T_priority=High  T=0 degC  T_nominal_specify=off  T_nominal_value=1  T_nominal_unit=K  Q_specify=off  Q_priority=None  Q=0 W  Q_nominal_specify=off  Q_nominal_value=1  Q_nominal_unit=W
  G : PMIOPort  Side=Left
  C : PMIOPort  Port=2  Side=Left
  E : PMIOPort  Port=3  Side=Right
  tag scope: diode_HA_temp_Q3=scoped, diode_JH_temp_Q3=scoped, diode_current_Q3=scoped, diode_ploss_Q3=scoped, igbt_HA_temp_Q3=scoped, igbt_JH_temp_Q3=scoped, igbt_current_Q3=scoped, igbt_ploss_Q3=scoped
  wires:
  PS-Simulink Converter3/1 -> [igbt_HA_temp_Q3]  "igbt_HA_temp"
  PS-Simulink Converter4/1 -> [igbt_ploss_Q3]  "Power Losses"
  PS-Simulink Converter2/1 -> [igbt_JH_temp_Q3]  "igbt_JH_temp"
  PS-Simulink Converter1/1 -> [diode_ploss_Q3]  "Power Losses"
  PS-Simulink Converter5/1 -> [diode_JH_temp_Q3]  "igbt_JH_temp"
  PS-Simulink Converter6/1 -> [diode_HA_temp_Q3]  "igbt_HA_temp"
  iph1/1 -> [igbt_current_Q3]  "i_device_thermal_inv"
  iph2/1 -> [diode_current_Q3]  "i_device_thermal_inv"
  connections:
  Temperature Sensor/RConn2 -- PS-Simulink Converter2/LConn1
  "IGBT_SIMPLE_2TH Simplified IGBT + antiparallel FWD, separate thermal ports"/LConn2 -- junction_thermal_mass_t/LConn1 -- power_losses_switch/LConn1
  Temperature Sensor1/RConn2 -- PS-Simulink Converter3/LConn1
  switch_heatsink/LConn1 -- heatsink_C/LConn1 -- switch_sandwich/RConn1 -- Temperature Sensor1/LConn1 -- Temperature Sensor/RConn1
  switch_heatsink/RConn1 -- Tambient/LConn1 -- Temperature Sensor1/RConn1
  switch_sandwich/LConn1 -- power_losses_switch/RConn2 -- Temperature Sensor/LConn1
  "IGBT_SIMPLE_2TH Simplified IGBT + antiparallel FWD, separate thermal ports"/RConn1 -- E/RConn1
  "IGBT_SIMPLE_2TH Simplified IGBT + antiparallel FWD, separate thermal ports"/LConn1 -- C/RConn1
  "IGBT_SIMPLE_2TH Simplified IGBT + antiparallel FWD, separate thermal ports"/LConn3 -- G/RConn1
  Temperature Sensor2/RConn1 -- Temperature Sensor3/LConn1 -- heatsink_C1/LConn1 -- switch_heatsink1/LConn1 -- switch_sandwich1/RConn1
  Tambient1/LConn1 -- switch_heatsink1/RConn1 -- Temperature Sensor3/RConn1
  power_losses_switch1/RConn2 -- switch_sandwich1/LConn1 -- Temperature Sensor2/LConn1
  Temperature Sensor3/RConn2 -- PS-Simulink Converter6/LConn1
  Temperature Sensor2/RConn2 -- PS-Simulink Converter5/LConn1
  power_losses_switch1/LConn1 -- junction_thermal_mass_d/LConn1 -- "IGBT_SIMPLE_2TH Simplified IGBT + antiparallel FWD, separate thermal ports"/RConn2
  iph1/LConn1 -- "IGBT_SIMPLE_2TH Simplified IGBT + antiparallel FWD, separate thermal ports"/RConn5
  iph2/LConn1 -- "IGBT_SIMPLE_2TH Simplified IGBT + antiparallel FWD, separate thermal ports"/RConn6
  "IGBT_SIMPLE_2TH Simplified IGBT + antiparallel FWD, separate thermal ports"/RConn3 -- PS Terminator/LConn1
  "IGBT_SIMPLE_2TH Simplified IGBT + antiparallel FWD, separate thermal ports"/RConn4 -- PS Terminator1/LConn1
  PS-Simulink Converter1/LConn1 -- power_losses_switch1/RConn1
  PS-Simulink Converter4/LConn1 -- power_losses_switch/RConn1
